simulink model "fix_FOC_sync"  (R2025b)
settings: Solver=FixedStepAuto  StartTime=0.0  StopTime=10.0  FixedStep=0.001  RelTol=1e-3
values from neighbouring files (symbols this model uses):
  Dm = 1e-3    (= 0.001)    [motor_param.m]
  Ki_id = wc_c*Rs    (= 380)    [motor_param.m]
  Ki_iq = wc_c*Rs    (= 380)    [motor_param.m]
  Ki_s = 0.041    [motor_param.m]
  Kp_id = wc_c*Ld    (= 10)    [motor_param.m]
  Kp_iq = wc_c*Lq    (= 20)    [motor_param.m]
  Kp_s = 0.0014    [motor_param.m]
  Ld = 0.01    [motor_param.m]
  Lq = 0.02    [motor_param.m]
  p = 2    [motor_param.m]
  Phi = 0.1    [motor_param.m]
libraries: fl_lib x50, nesl_utility x50, slpidlib x15, ee_lib x15, eeTransforms x10
(part 4 of 4)

== system fix_FOC_sync/Subsystem4/Controller/FOC/VelocityController ==
  wmref : Inport
  wm : Inport  Port=2
  Gain : Gain  Gain=1/(3/2*p*Phi)
  PIDController : slpidlib/PID Controller  Controller=PI  Form=Parallel  TimeDomain=Continuous-time  UseExternalTs=off  SampleTime=-1  IntegratorMethod=Forward Euler  FilterMethod=Forward Euler  ControllerParametersSource=internal  P=Kp_s  I=Ki_s  UseKiTs=off  D=0  UseExternalDerivativeSource=off  N=100  UseFilter=on  TunerSelectOption=Transfer Function Based (PID Tuner App)  InitialConditionSource=internal  InitialConditionForIntegrator=0  InitialConditionForFilter=0  DifferentiatorICPrevScaledInput=0  ExternalReset=none  TrackingMode=off  Kt=1  LimitOutput=off  SatLimitsSource=internal  UpperSaturationLimit=inf  LowerSaturationLimit=-inf  LinearizeAsGain=on  AntiWindupMode=none  Kb=1  LimitIntegrator=off  UpperIntegratorSaturationLimit=inf  LowerIntegratorSaturationLimit=-inf  POutMin=[]  POutMax=[]  IOutMin=[]  IOutMax=[]  DOutMin=[]  DOutMax=[]  NOutMin=[]  NOutMax=[]  SumOutMin=[]  SumOutMax=[]  SaturationOutMin=[]  SaturationOutMax=[]  PParamMin=[]  PParamMax=[]  IParamMin=[]  IParamMax=[]  DParamMin=[]  DParamMax=[]  NParamMin=[]  NParamMax=[]  KbParamMin=[]  KbParamMax=[]  KtParamMin=[]  KtParamMax=[]  KbOutMin=[]  KbOutMax=[]  KtOutMin=[]  KtOutMax=[]  IntegratorOutMin=[]  IntegratorOutMax=[]  FilterOutMin=[]  FilterOutMax=[]  SumI1OutMin=[]  SumI1OutMax=[]  SumI2OutMin=[]  SumI2OutMax=[]  SumI3OutMin=[]  SumI3OutMax=[]  SumI4OutMin=[]  SumI4OutMax=[]  SumDOutMin=[]  SumDOutMax=[]  DifferentiatorOutMin=[]  DifferentiatorOutMax=[]  FilterDiffOutCoefMin=[]  FilterDiffOutCoefMax=[]  ReciprocalOutMin=[]  ReciprocalOutMax=[]  SumDenOutMin=[]  SumDenOutMax=[]  SumNumOutMin=[]  SumNumOutMax=[]  DivideOutMin=[]  DivideOutMax=[]  UdiffTsProdOutMin=[]  UdiffTsProdOutMax=[]  NTsProdOutMin=[]  NTsProdOutMax=[]  UintegralTsProdOutMin=[]  UintegralTsProdOutMax=[]  UngainTsProdOutMin=[]  UngainTsProdOutMax=[]  ClampingZeroOutDataTypeStr=Inherit: Inherit via back propagation  ClampingZeroOutMin=[]  ClampingZeroOutMax=[]  FilterDenConstantOutDataTypeStr=Inherit: Inherit via back propagation  FilterDenConstantOutMin=[]  FilterDenConstantOutMax=[]  PCopyOutDataTypeStr=Inherit: Inherit via back propagation  PCopyOutMin=[]  PCopyOutMax=[]  NCopyOutDataTypeStr=Inherit: Inherit via back propagation  NCopyOutMin=[]  NCopyOutMax=[]  IntegratorContinuousStateAttributes=''  IntegratorStateMustResolveToSignalObject=off  IntegratorRTWStateStorageClass=Auto  FilterContinuousStateAttributes=''  FilterStateMustResolveToSignalObject=off  FilterRTWStateStorageClass=Auto  ParallelPVariant=InternalParameters  IdealPVariant=Disabled  IVariant=InternalParameters  DVariant=Disabled  IntegratorVariant=Continuous  SatVariant=Disabled  AWVariant=Passthrough  PCopyVariant=Disabled  TRVariant=Disabled  FdbkBlocksVariant=Forward  IdealPFdbkVariant=Disabled  SatFdbkVariant=Disabled  DerivativeFilterVariant=Disabled  NVariant=Disabled  NCopyVariant=Disabled_SignalSpec  FilterICVariant=Disabled  IntegratorICVariant=InternalICs  ExternalResetVariant=Disabled  TRSumVariant=Passthrough  SumFdbkVariant=Disabled  SumVariant=Sum_PI  TsampFilterVariant=InternalTs  TsampNgainVariant=Passthrough  TsampIntegralVariant=Disabled_SignalSpec  ExternalSaturationOutDataTypeStr=Inherit: Same as second input  DerivativeSourceVariant=Disabled  PreIntVariant=InternalPreInt
  Sum : Sum  Inputs=|+-
  Iqref : Outport  VectorParamsAs1DForOutWhenUnconnected=off
  wires:
  PIDController/1 -> Gain/1
  Gain/1 -> Iqref/1
  wmref/1 -> Sum/1
  Sum/1 -> PIDController/1
  wm/1 -> Sum/2

== system fix_FOC_sync/Subsystem4/Controller/FOC/abc2dq ==
  Iabc : Inport
  thetae : Inport  Port=2
  Demux1 : Demux  Outputs=3
  Park Transform : eeTransforms/Park Transform  AxisAlignment=D-axis  PowerInvariant=off
  Terminator : Terminator
  Id : Outport  VectorParamsAs1DForOutWhenUnconnected=off
  Iq : Outport  Port=2  VectorParamsAs1DForOutWhenUnconnected=off
  wires:
  Iabc/1 -> Park Transform/1
  thetae/1 -> Park Transform/2
  Demux1/3 -> Terminator/1
  Park Transform/1 -> Demux1/1
  Demux1/1 -> Id/1
  Demux1/2 -> Iq/1

== system fix_FOC_sync/Subsystem4/Controller/FOC/dq2abc ==
  Vd : Inport
  Vq : Inport  Port=2
  thetae : Inport  Port=3
  Constant : Constant  Value=0
  Inverse Park Transform : eeTransforms/Inverse Park Transform  AxisAlignment=D-axis  PowerInvariant=off
  Mux : Mux  Inputs=3
  Vabc : Outport  VectorParamsAs1DForOutWhenUnconnected=off
  wires:
  thetae/1 -> Inverse Park Transform/2
  Constant/1 -> Mux/3
  Mux/1 -> Inverse Park Transform/1
  Vd/1 -> Mux/1
  Inverse Park Transform/1 -> Vabc/1
  Vq/1 -> Mux/2

== system fix_FOC_sync/Subsystem4/Controller/FOC/thm2the ==
  thm : Inport
  Constant : Constant  Value=2*pi
  Mod : Math  Operator=mod  SignedPower=on
  PolePairs : Gain  Gain=p
  the : Outport  VectorParamsAs1DForOutWhenUnconnected=off
  wires:
  Constant/1 -> Mod/2
  PolePairs/1 -> Mod/1
  Mod/1 -> the/1
  thm/1 -> PolePairs/1

== system fix_FOC_sync/Subsystem4/Controller/FOC/wm2we ==
  wm : Inport
  PolePairs : Gain  Gain=p
  we : Outport  VectorParamsAs1DForOutWhenUnconnected=off
  wires:
  wm/1 -> PolePairs/1
  PolePairs/1 -> we/1

== system fix_FOC_sync/Subsystem5/Controller/DriverPeripherals/Break Algebraic Loop ==
  In1 : Inport
  Demux : Demux  Outputs=3
  Mux : Mux  Inputs=3
  Transfer Fcn : TransferFcn  Denominator=[1e-6 1]
  Transfer Fcn1 : TransferFcn  Denominator=[1e-6 1]
  Transfer Fcn2 : TransferFcn  Denominator=[1e-6 1]
  Out1 : Outport
  wires:
  In1/1 -> Demux/1
  Demux/1 -> Transfer Fcn/1
  Transfer Fcn/1 -> Mux/1
  Demux/2 -> Transfer Fcn1/1
  Transfer Fcn1/1 -> Mux/2
  Demux/3 -> Transfer Fcn2/1
  Transfer Fcn2/1 -> Mux/3
  Mux/1 -> Out1/1

== system fix_FOC_sync/Subsystem5/Controller/FOC/CurrentController ==
  Idref : Inport
  Iqref : Inport  Port=2
  Id : Inport  Port=3
  Iq : Inport  Port=4
  we : Inport  Port=5
  Decoupling : Subsystem
  IdController : slpidlib/PID Controller  Controller=PI  Form=Parallel  TimeDomain=Continuous-time  UseExternalTs=off  SampleTime=-1  IntegratorMethod=Forward Euler  FilterMethod=Forward Euler  ControllerParametersSource=internal  P=Kp_id  I=Ki_id  UseKiTs=off  D=0  UseExternalDerivativeSource=off  N=100  UseFilter=on  TunerSelectOption=Transfer Function Based (PID Tuner App)  InitialConditionSource=internal  InitialConditionForIntegrator=0  InitialConditionForFilter=0  DifferentiatorICPrevScaledInput=0  ExternalReset=none  TrackingMode=off  Kt=1  LimitOutput=off  SatLimitsSource=internal  UpperSaturationLimit=inf  LowerSaturationLimit=-inf  LinearizeAsGain=on  AntiWindupMode=none  Kb=1  LimitIntegrator=off  UpperIntegratorSaturationLimit=inf  LowerIntegratorSaturationLimit=-inf  POutMin=[]  POutMax=[]  IOutMin=[]  IOutMax=[]  DOutMin=[]  DOutMax=[]  NOutMin=[]  NOutMax=[]  SumOutMin=[]  SumOutMax=[]  SaturationOutMin=[]  SaturationOutMax=[]  PParamMin=[]  PParamMax=[]  IParamMin=[]  IParamMax=[]  DParamMin=[]  DParamMax=[]  NParamMin=[]  NParamMax=[]  KbParamMin=[]  KbParamMax=[]  KtParamMin=[]  KtParamMax=[]  KbOutMin=[]  KbOutMax=[]  KtOutMin=[]  KtOutMax=[]  IntegratorOutMin=[]  IntegratorOutMax=[]  FilterOutMin=[]  FilterOutMax=[]  SumI1OutMin=[]  SumI1OutMax=[]  SumI2OutMin=[]  SumI2OutMax=[]  SumI3OutMin=[]  SumI3OutMax=[]  SumI4OutMin=[]  SumI4OutMax=[]  SumDOutMin=[]  SumDOutMax=[]  DifferentiatorOutMin=[]  DifferentiatorOutMax=[]  FilterDiffOutCoefMin=[]  FilterDiffOutCoefMax=[]  ReciprocalOutMin=[]  ReciprocalOutMax=[]  SumDenOutMin=[]  SumDenOutMax=[]  SumNumOutMin=[]  SumNumOutMax=[]  DivideOutMin=[]  DivideOutMax=[]  UdiffTsProdOutMin=[]  UdiffTsProdOutMax=[]  NTsProdOutMin=[]  NTsProdOutMax=[]  UintegralTsProdOutMin=[]  UintegralTsProdOutMax=[]  UngainTsProdOutMin=[]  UngainTsProdOutMax=[]  ClampingZeroOutDataTypeStr=Inherit: Inherit via back propagation  ClampingZeroOutMin=[]  ClampingZeroOutMax=[]  FilterDenConstantOutDataTypeStr=Inherit: Inherit via back propagation  FilterDenConstantOutMin=[]  FilterDenConstantOutMax=[]  PCopyOutDataTypeStr=Inherit: Inherit via back propagation  PCopyOutMin=[]  PCopyOutMax=[]  NCopyOutDataTypeStr=Inherit: Inherit via back propagation  NCopyOutMin=[]  NCopyOutMax=[]  IntegratorContinuousStateAttributes=''  IntegratorStateMustResolveToSignalObject=off  IntegratorRTWStateStorageClass=Auto  FilterContinuousStateAttributes=''  FilterStateMustResolveToSignalObject=off  FilterRTWStateStorageClass=Auto  ParallelPVariant=InternalParameters  IdealPVariant=Disabled  IVariant=InternalParameters  DVariant=Disabled  IntegratorVariant=Continuous  SatVariant=Disabled  AWVariant=Passthrough  PCopyVariant=Disabled  TRVariant=Disabled  FdbkBlocksVariant=Forward  IdealPFdbkVariant=Disabled  SatFdbkVariant=Disabled  DerivativeFilterVariant=Disabled  NVariant=Disabled  NCopyVariant=Disabled_SignalSpec  FilterICVariant=Disabled  IntegratorICVariant=InternalICs  ExternalResetVariant=Disabled  TRSumVariant=Passthrough  SumFdbkVariant=Disabled  SumVariant=Sum_PI  TsampFilterVariant=InternalTs  TsampNgainVariant=Passthrough  TsampIntegralVariant=Disabled_SignalSpec  ExternalSaturationOutDataTypeStr=Inherit: Same as second input  DerivativeSourceVariant=Disabled  PreIntVariant=InternalPreInt
  IqController : slpidlib/PID Controller  Controller=PI  Form=Parallel  TimeDomain=Continuous-time  UseExternalTs=off  SampleTime=-1  IntegratorMethod=Forward Euler  FilterMethod=Forward Euler  ControllerParametersSource=internal  P=Kp_iq  I=Ki_iq  UseKiTs=off  D=0  UseExternalDerivativeSource=off  N=100  UseFilter=on  TunerSelectOption=Transfer Function Based (PID Tuner App)  InitialConditionSource=internal  InitialConditionForIntegrator=0  InitialConditionForFilter=0  DifferentiatorICPrevScaledInput=0  ExternalReset=none  TrackingMode=off  Kt=1  LimitOutput=off  SatLimitsSource=internal  UpperSaturationLimit=inf  LowerSaturationLimit=-inf  LinearizeAsGain=on  AntiWindupMode=none  Kb=1  LimitIntegrator=off  UpperIntegratorSaturationLimit=inf  LowerIntegratorSaturationLimit=-inf  POutMin=[]  POutMax=[]  IOutMin=[]  IOutMax=[]  DOutMin=[]  DOutMax=[]  NOutMin=[]  NOutMax=[]  SumOutMin=[]  SumOutMax=[]  SaturationOutMin=[]  SaturationOutMax=[]  PParamMin=[]  PParamMax=[]  IParamMin=[]  IParamMax=[]  DParamMin=[]  DParamMax=[]  NParamMin=[]  NParamMax=[]  KbParamMin=[]  KbParamMax=[]  KtParamMin=[]  KtParamMax=[]  KbOutMin=[]  KbOutMax=[]  KtOutMin=[]  KtOutMax=[]  IntegratorOutMin=[]  IntegratorOutMax=[]  FilterOutMin=[]  FilterOutMax=[]  SumI1OutMin=[]  SumI1OutMax=[]  SumI2OutMin=[]  SumI2OutMax=[]  SumI3OutMin=[]  SumI3OutMax=[]  SumI4OutMin=[]  SumI4OutMax=[]  SumDOutMin=[]  SumDOutMax=[]  DifferentiatorOutMin=[]  DifferentiatorOutMax=[]  FilterDiffOutCoefMin=[]  FilterDiffOutCoefMax=[]  ReciprocalOutMin=[]  ReciprocalOutMax=[]  SumDenOutMin=[]  SumDenOutMax=[]  SumNumOutMin=[]  SumNumOutMax=[]  DivideOutMin=[]  DivideOutMax=[]  UdiffTsProdOutMin=[]  UdiffTsProdOutMax=[]  NTsProdOutMin=[]  NTsProdOutMax=[]  UintegralTsProdOutMin=[]  UintegralTsProdOutMax=[]  UngainTsProdOutMin=[]  UngainTsProdOutMax=[]  ClampingZeroOutDataTypeStr=Inherit: Inherit via back propagation  ClampingZeroOutMin=[]  ClampingZeroOutMax=[]  FilterDenConstantOutDataTypeStr=Inherit: Inherit via back propagation  FilterDenConstantOutMin=[]  FilterDenConstantOutMax=[]  PCopyOutDataTypeStr=Inherit: Inherit via back propagation  PCopyOutMin=[]  PCopyOutMax=[]  NCopyOutDataTypeStr=Inherit: Inherit via back propagation  NCopyOutMin=[]  NCopyOutMax=[]  IntegratorContinuousStateAttributes=''  IntegratorStateMustResolveToSignalObject=off  IntegratorRTWStateStorageClass=Auto  FilterContinuousStateAttributes=''  FilterStateMustResolveToSignalObject=off  FilterRTWStateStorageClass=Auto  ParallelPVariant=InternalParameters  IdealPVariant=Disabled  IVariant=InternalParameters  DVariant=Disabled  IntegratorVariant=Continuous  SatVariant=Disabled  AWVariant=Passthrough  PCopyVariant=Disabled  TRVariant=Disabled  FdbkBlocksVariant=Forward  IdealPFdbkVariant=Disabled  SatFdbkVariant=Disabled  DerivativeFilterVariant=Disabled  NVariant=Disabled  NCopyVariant=Disabled_SignalSpec  FilterICVariant=Disabled  IntegratorICVariant=InternalICs  ExternalResetVariant=Disabled  TRSumVariant=Passthrough  SumFdbkVariant=Disabled  SumVariant=Sum_PI  TsampFilterVariant=InternalTs  TsampNgainVariant=Passthrough  TsampIntegralVariant=Disabled_SignalSpec  ExternalSaturationOutDataTypeStr=Inherit: Same as second input  DerivativeSourceVariant=Disabled  PreIntVariant=InternalPreInt
  Sum1 : Sum  Inputs=|+-
  Sum2 : Sum  Inputs=++|
  Sum3 : Sum  Inputs=++|
  Sum4 : Sum  Inputs=|+-
  Vdref : Outport  VectorParamsAs1DForOutWhenUnconnected=off
  Vqref : Outport  Port=2  VectorParamsAs1DForOutWhenUnconnected=off
  wires:
  we/1 -> Decoupling/3(we)
  Idref/1 -> Sum4/1
  Sum2/1 -> Vdref/1
  Sum3/1 -> Vqref/1
  Iqref/1 -> Sum1/1
  Iq/1 -> Decoupling/2(Iq), Sum1/2
  Id/1 -> Decoupling/1(Id), Sum4/2
  Sum4/1 -> IdController/1
  Sum1/1 -> IqController/1
  Decoupling/2(VqFF) -> Sum3/1
  Decoupling/1(VdFF) -> Sum2/1
  IdController/1 -> Sum2/2
  IqController/1 -> Sum3/2

== system fix_FOC_sync/Subsystem5/Controller/FOC/VelocityController ==
  wmref : Inport
  wm : Inport  Port=2
  Gain : Gain  Gain=1/(3/2*p*Phi)
  PIDController : slpidlib/PID Controller  Controller=PI  Form=Parallel  TimeDomain=Continuous-time  UseExternalTs=off  SampleTime=-1  IntegratorMethod=Forward Euler  FilterMethod=Forward Euler  ControllerParametersSource=internal  P=Kp_s  I=Ki_s  UseKiTs=off  D=0  UseExternalDerivativeSource=off  N=100  UseFilter=on  TunerSelectOption=Transfer Function Based (PID Tuner App)  InitialConditionSource=internal  InitialConditionForIntegrator=0  InitialConditionForFilter=0  DifferentiatorICPrevScaledInput=0  ExternalReset=none  TrackingMode=off  Kt=1  LimitOutput=off  SatLimitsSource=internal  UpperSaturationLimit=inf  LowerSaturationLimit=-inf  LinearizeAsGain=on  AntiWindupMode=none  Kb=1  LimitIntegrator=off  UpperIntegratorSaturationLimit=inf  LowerIntegratorSaturationLimit=-inf  POutMin=[]  POutMax=[]  IOutMin=[]  IOutMax=[]  DOutMin=[]  DOutMax=[]  NOutMin=[]  NOutMax=[]  SumOutMin=[]  SumOutMax=[]  SaturationOutMin=[]  SaturationOutMax=[]  PParamMin=[]  PParamMax=[]  IParamMin=[]  IParamMax=[]  DParamMin=[]  DParamMax=[]  NParamMin=[]  NParamMax=[]  KbParamMin=[]  KbParamMax=[]  KtParamMin=[]  KtParamMax=[]  KbOutMin=[]  KbOutMax=[]  KtOutMin=[]  KtOutMax=[]  IntegratorOutMin=[]  IntegratorOutMax=[]  FilterOutMin=[]  FilterOutMax=[]  SumI1OutMin=[]  SumI1OutMax=[]  SumI2OutMin=[]  SumI2OutMax=[]  SumI3OutMin=[]  SumI3OutMax=[]  SumI4OutMin=[]  SumI4OutMax=[]  SumDOutMin=[]  SumDOutMax=[]  DifferentiatorOutMin=[]  DifferentiatorOutMax=[]  FilterDiffOutCoefMin=[]  FilterDiffOutCoefMax=[]  ReciprocalOutMin=[]  ReciprocalOutMax=[]  SumDenOutMin=[]  SumDenOutMax=[]  SumNumOutMin=[]  SumNumOutMax=[]  DivideOutMin=[]  DivideOutMax=[]  UdiffTsProdOutMin=[]  UdiffTsProdOutMax=[]  NTsProdOutMin=[]  NTsProdOutMax=[]  UintegralTsProdOutMin=[]  UintegralTsProdOutMax=[]  UngainTsProdOutMin=[]  UngainTsProdOutMax=[]  ClampingZeroOutDataTypeStr=Inherit: Inherit via back propagation  ClampingZeroOutMin=[]  ClampingZeroOutMax=[]  FilterDenConstantOutDataTypeStr=Inherit: Inherit via back propagation  FilterDenConstantOutMin=[]  FilterDenConstantOutMax=[]  PCopyOutDataTypeStr=Inherit: Inherit via back propagation  PCopyOutMin=[]  PCopyOutMax=[]  NCopyOutDataTypeStr=Inherit: Inherit via back propagation  NCopyOutMin=[]  NCopyOutMax=[]  IntegratorContinuousStateAttributes=''  IntegratorStateMustResolveToSignalObject=off  IntegratorRTWStateStorageClass=Auto  FilterContinuousStateAttributes=''  FilterStateMustResolveToSignalObject=off  FilterRTWStateStorageClass=Auto  ParallelPVariant=InternalParameters  IdealPVariant=Disabled  IVariant=InternalParameters  DVariant=Disabled  IntegratorVariant=Continuous  SatVariant=Disabled  AWVariant=Passthrough  PCopyVariant=Disabled  TRVariant=Disabled  FdbkBlocksVariant=Forward  IdealPFdbkVariant=Disabled  SatFdbkVariant=Disabled  DerivativeFilterVariant=Disabled  NVariant=Disabled  NCopyVariant=Disabled_SignalSpec  FilterICVariant=Disabled  IntegratorICVariant=InternalICs  ExternalResetVariant=Disabled  TRSumVariant=Passthrough  SumFdbkVariant=Disabled  SumVariant=Sum_PI  TsampFilterVariant=InternalTs  TsampNgainVariant=Passthrough  TsampIntegralVariant=Disabled_SignalSpec  ExternalSaturationOutDataTypeStr=Inherit: Same as second input  DerivativeSourceVariant=Disabled  PreIntVariant=InternalPreInt
  Sum : Sum  Inputs=|+-
  Iqref : Outport  VectorParamsAs1DForOutWhenUnconnected=off
  wires:
  PIDController/1 -> Gain/1
  Gain/1 -> Iqref/1
  wmref/1 -> Sum/1
  Sum/1 -> PIDController/1
  wm/1 -> Sum/2

== system fix_FOC_sync/Subsystem5/Controller/FOC/abc2dq ==
  Iabc : Inport
  thetae : Inport  Port=2
  Demux1 : Demux  Outputs=3
  Park Transform : eeTransforms/Park Transform  AxisAlignment=D-axis  PowerInvariant=off
  Terminator : Terminator
  Id : Outport  VectorParamsAs1DForOutWhenUnconnected=off
  Iq : Outport  Port=2  VectorParamsAs1DForOutWhenUnconnected=off
  wires:
  Iabc/1 -> Park Transform/1
  thetae/1 -> Park Transform/2
  Demux1/3 -> Terminator/1
  Park Transform/1 -> Demux1/1
  Demux1/1 -> Id/1
  Demux1/2 -> Iq/1

== system fix_FOC_sync/Subsystem5/Controller/FOC/dq2abc ==
  Vd : Inport
  Vq : Inport  Port=2
  thetae : Inport  Port=3
  Constant : Constant  Value=0
  Inverse Park Transform : eeTransforms/Inverse Park Transform  AxisAlignment=D-axis  PowerInvariant=off
  Mux : Mux  Inputs=3
  Vabc : Outport  VectorParamsAs1DForOutWhenUnconnected=off
  wires:
  thetae/1 -> Inverse Park Transform/2
  Constant/1 -> Mux/3
  Mux/1 -> Inverse Park Transform/1
  Vd/1 -> Mux/1
  Inverse Park Transform/1 -> Vabc/1
  Vq/1 -> Mux/2

== system fix_FOC_sync/Subsystem5/Controller/FOC/thm2the ==
  thm : Inport
  Constant : Constant  Value=2*pi
  Mod : Math  Operator=mod  SignedPower=on
  PolePairs : Gain  Gain=p
  the : Outport  VectorParamsAs1DForOutWhenUnconnected=off
  wires:
  Constant/1 -> Mod/2
  PolePairs/1 -> Mod/1
  Mod/1 -> the/1
  thm/1 -> PolePairs/1

== system fix_FOC_sync/Subsystem5/Controller/FOC/wm2we ==
  wm : Inport
  PolePairs : Gain  Gain=p
  we : Outport  VectorParamsAs1DForOutWhenUnconnected=off
  wires:
  wm/1 -> PolePairs/1
  PolePairs/1 -> we/1

== system fix_FOC_sync/Subsystem1/Controller/FOC/CurrentController/Decoupling ==
  note: VdFF = -Lq*Iq*we
  note: VqFF = Ld*Id*we + Phi*we
  Id : Inport
  Iq : Inport  Port=2
  we : Inport  Port=3
  Constant : Constant  Value=Lq
  Constant1 : Constant  Value=Ld
  Constant2 : Constant  Value=Phi
  Gain1 : Gain  Gain=-1
  Product{,1..3} (4 alike) : Product
  Sum : Sum  Inputs=|++
  VdFF : Outport  VectorParamsAs1DForOutWhenUnconnected=off
  VqFF : Outport  Port=2  VectorParamsAs1DForOutWhenUnconnected=off
  wires:
  we/1 -> Product3/2, Product2/2
  Product1/1 -> Sum/1
  Constant2/1 -> Sum/2
  Sum/1 -> Product2/1
  Constant1/1 -> Product1/2
  Id/1 -> Product1/1
  Iq/1 -> Product/1
  Constant/1 -> Product/2
  Product3/1 -> Gain1/1
  Product/1 -> Product3/1
  Gain1/1 -> VdFF/1
  Product2/1 -> VqFF/1

== system fix_FOC_sync/Subsystem2/Controller/FOC/CurrentController/Decoupling ==
  note: VdFF = -Lq*Iq*we
  note: VqFF = Ld*Id*we + Phi*we
  Id : Inport
  Iq : Inport  Port=2
  we : Inport  Port=3
  Constant : Constant  Value=Lq
  Constant1 : Constant  Value=Ld
  Constant2 : Constant  Value=Phi
  Gain1 : Gain  Gain=-1
  Product{,1..3} (4 alike) : Product
  Sum : Sum  Inputs=|++
  VdFF : Outport  VectorParamsAs1DForOutWhenUnconnected=off
  VqFF : Outport  Port=2  VectorParamsAs1DForOutWhenUnconnected=off
  wires:
  we/1 -> Product3/2, Product2/2
  Product1/1 -> Sum/1
  Constant2/1 -> Sum/2
  Sum/1 -> Product2/1
  Constant1/1 -> Product1/2
  Id/1 -> Product1/1
  Iq/1 -> Product/1
  Constant/1 -> Product/2
  Product3/1 -> Gain1/1
  Product/1 -> Product3/1
  Gain1/1 -> VdFF/1
  Product2/1 -> VqFF/1

== system fix_FOC_sync/Subsystem3/Controller/FOC/CurrentController/Decoupling ==
  note: VdFF = -Lq*Iq*we
  note: VqFF = Ld*Id*we + Phi*we
  Id : Inport
  Iq : Inport  Port=2
  we : Inport  Port=3
  Constant : Constant  Value=Lq
  Constant1 : Constant  Value=Ld
  Constant2 : Constant  Value=Phi
  Gain1 : Gain  Gain=-1
  Product{,1..3} (4 alike) : Product
  Sum : Sum  Inputs=|++
  VdFF : Outport  VectorParamsAs1DForOutWhenUnconnected=off
  VqFF : Outport  Port=2  VectorParamsAs1DForOutWhenUnconnected=off
  wires:
  we/1 -> Product3/2, Product2/2
  Product1/1 -> Sum/1
  Constant2/1 -> Sum/2
  Sum/1 -> Product2/1
  Constant1/1 -> Product1/2
  Id/1 -> Product1/1
  Iq/1 -> Product/1
  Constant/1 -> Product/2
  Product3/1 -> Gain1/1
  Product/1 -> Product3/1
  Gain1/1 -> VdFF/1
  Product2/1 -> VqFF/1

== system fix_FOC_sync/Subsystem4/Controller/FOC/CurrentController/Decoupling ==
  note: VdFF = -Lq*Iq*we
  note: VqFF = Ld*Id*we + Phi*we
  Id : Inport
  Iq : Inport  Port=2
  we : Inport  Port=3
  Constant : Constant  Value=Lq
  Constant1 : Constant  Value=Ld
  Constant2 : Constant  Value=Phi
  Gain1 : Gain  Gain=-1
  Product{,1..3} (4 alike) : Product
  Sum : Sum  Inputs=|++
  VdFF : Outport  VectorParamsAs1DForOutWhenUnconnected=off
  VqFF : Outport  Port=2  VectorParamsAs1DForOutWhenUnconnected=off
  wires:
  we/1 -> Product3/2, Product2/2
  Product1/1 -> Sum/1
  Constant2/1 -> Sum/2
  Sum/1 -> Product2/1
  Constant1/1 -> Product1/2
  Id/1 -> Product1/1
  Iq/1 -> Product/1
  Constant/1 -> Product/2
  Product3/1 -> Gain1/1
  Product/1 -> Product3/1
  Gain1/1 -> VdFF/1
  Product2/1 -> VqFF/1

== system fix_FOC_sync/Subsystem5/Controller/FOC/CurrentController/Decoupling ==
  note: VdFF = -Lq*Iq*we
  note: VqFF = Ld*Id*we + Phi*we
  Id : Inport
  Iq : Inport  Port=2
  we : Inport  Port=3
  Constant : Constant  Value=Lq
  Constant1 : Constant  Value=Ld
  Constant2 : Constant  Value=Phi
  Gain1 : Gain  Gain=-1
  Product{,1..3} (4 alike) : Product
  Sum : Sum  Inputs=|++
  VdFF : Outport  VectorParamsAs1DForOutWhenUnconnected=off
  VqFF : Outport  Port=2  VectorParamsAs1DForOutWhenUnconnected=off
  wires:
  we/1 -> Product3/2, Product2/2
  Product1/1 -> Sum/1
  Constant2/1 -> Sum/2
  Sum/1 -> Product2/1
  Constant1/1 -> Product1/2
  Id/1 -> Product1/1
  Iq/1 -> Product/1
  Constant/1 -> Product/2
  Product3/1 -> Gain1/1
  Product/1 -> Product3/1
  Gain1/1 -> VdFF/1
  Product2/1 -> VqFF/1

== matlab function fix_FOC_sync/Subsystem6/MATLAB Function ==
  data: theta0 input; omega_cmd output; theta_meas input; om_hat input
function omega_cmd  = Controller(theta0, theta_meas, om_hat)
%#codegen
% 输入:
%   theta0     - 领导者角度（标量）
%   theta_meas - 5x1 电机角度（编码器）
%   om_hat     - 5x1 前馈（观测器估计的领导者角速度）
%   v_f        - 5x1 低通滤波状态（来自 Integrator）
% 输出:
%   omega_cmd  - 5x1 未滤波控制器输出（仅记录/监控）
%   dv_f       - 5x1 滤波状态导数（送 Integrator）

n = 5;
L = 2*eye(n) - diag(ones(n-1,1),1) - diag(ones(n-1,1),-1);
B = diag([1, 0, 1, 0, 0]);

p1 = 0.75;  p2 = 1.5;
k1 = 5;    k2 = 5;

tau_f = 1e-2;   % ★ 低通时间常数

sig = @(x,a) sign(x).*abs(x).^a;
th0 = theta0(1);   % 强制标量

omega_cmd = zeros(n,1);
for i = 1:n
    ei = 0;
    for j = 1:n
        if i ~= j && L(i,j) ~= 0
            ei = ei + (-L(i,j))*(theta_meas(i) - theta_meas(j));
        end
    end
    if B(i,i) == 1
        ei = ei + (theta_meas(i) - th0);
    end
    omega_cmd(i) = min(max(om_hat(i) - k1*sig(ei,p1) - k2*sig(ei,p2),-50),50);
end


end

== matlab function fix_FOC_sync/Subsystem6/MATLAB Function4 ==
  data: dth_hat output; dom_hat output; theta0 input; th_hat input; om_hat input
%% ObserverRHS
function [dth_hat, dom_hat] = ObserverRHS(theta0, th_hat, om_hat)
%#codegen
n = 5;
L = 2*eye(n) - diag(ones(n-1,1),1) - diag(ones(n-1,1),-1);
B = diag([1, 0, 1, 0, 0]);

a1 = 0.7;  a2 = 1.3;
a3 = 2*a1-1;  a4 = 2*a2-1;
c1 = 50;  c2 = 50;     % ★ 加大
c3 = 500; c4 = 500;    % ★ 加大

sig = @(x,a) sign(x).*abs(x).^a;

th0 = theta0(1);       % ★ 强制标量

e = zeros(n,1);
for i = 1:n
    ei = 0;
    for j = 1:n
        if i ~= j && L(i,j) ~= 0
            ei = ei + (-L(i,j))*(th_hat(i) - th_hat(j));
        end
    end
    if B(i,i) == 1
        ei = ei + (th_hat(i) - th0);
    end
    e(i) = ei;
end

dth_hat = om_hat - c1*sig(e,a1) - c2*sig(e,a2);
dom_hat =          - c3*sig(e,a3) - c4*sig(e,a4);
end
